simulink model "unit_decide"  (R2026b)
settings: Solver=FixedStepDiscrete  EnableMultiTasking=on
values from neighbouring files (symbols this model uses):
  STALL_SEC = 1.0    [sign_detector.sldd]
  VOTE_K = 3.0    [sign_detector.sldd]
  VOTE_N = 5.0    [sign_detector.sldd]
settings Model: DataDictionary=sign_detector.sldd  Creator=don  LastModifiedBy=don
settings SolverCC: PositivePriorityOrder=on
settings OptimizationCC: DifferentSizesBufferReuse=on  EfficientFloat2IntCast=on  EfficientTunableParamExpr=on  EnhancedBackFolding=on  LifeSpan=Inf  MaxStackSize=200000  OptimizationCustomize=off  OptimizeBlockOrder=speed  PassReuseOutputArgsAs=Individual arguments  UseDivisionForNetSlopeComputation=on
settings DebuggingCC: AlgebraicLoopMsg=error  ArtificialAlgebraicLoopMsg=error  AssertControl=DisableAll  BlockPriorityViolationMsg=error  BusObjectLabelMismatch=error  CheckMatrixSingularityMsg=error  InheritedTsInSrcMsg=error  IntegerOverflowMsg=error  IntegerSaturationMsg=error  ModelReferenceDataLoggingMessage=error  ModelReferenceIOMismatchMessage=error  NonBusSignalsTreatedAsBus=error  ParameterPrecisionLossMsg=error  ParameterTunabilityLossMsg=error  ParameterUnderflowMsg=error  ReadBeforeWriteMsg=EnableAllAsError  RootOutportRequireBusObject=error  SFcnCompatibilityMsg=error  SaveWithDisabledLinksMsg=error  SaveWithParameterizedLinksMsg=error  SigSpecEnsureSampleTimeMsg=error  SignalInfNanChecking=error  SignalLabelMismatchMsg=error  SignalRangeChecking=error  SolverPrmCheckMsg=error  StateNameClashWarn=warning  StrictBusMsg=ErrorOnBusTreatedAsVector  TasksWithSamePriorityMsg=error  UnconnectedInputMsg=error  UnconnectedLineMsg=error  UnconnectedOutputMsg=error  UnderSpecifiedDataTypeMsg=error  UniqueDataStoreMsg=error  UnknownTsInhSupMsg=error  UnnecessaryDatatypeConvMsg=warning  VariantConditionMismatch=error  VectorMatrixConversionMsg=error  WriteAfterReadMsg=EnableAllAsError  WriteAfterWriteMsg=EnableAllAsError
settings HardwareCC: ProdHWDeviceType=ARM Compatible->ARM Cortex-A (64-bit)  ProdLargestAtomicFloat=Double  ProdLargestAtomicInteger=LongLong  ProdLongLongMode=on
settings ModelReferenceCC: ModelReferenceNumInstancesAllowed=Single
settings SFSimCC: EnableRuntimeRecursion=off  MATLABDynamicMemAlloc=off
settings RTWCC: BuildConfiguration=Faster Runs  Description=Embedded Coder  HardwareBoard=Raspberry Pi (64bit)  SystemTargetFile=ert.tlc  TLCOptions="-aInlineSetEventsForThisBaseRateFcn=TLC_FALSE -aSuppressMultiTaskScheduler=TLC_FALSE  -aRateBasedStepFcn=0"  TargetLang=C++  TemplateMakefile=ert_default_tmf  Toolchain=GNU GCC RPIUtils
settings CodeAppCC: ForceParamTrailComments=on  IgnoreCustomStorageClasses=off  InsertBlockDesc=on  MATLABFcnDesc=on  MATLABSourceComments=on  OperatorAnnotations=on  ReqsInCode=on  SFDataObjDesc=on  SimulinkDataObjDesc=on  StateflowObjectComments=on
settings ERTTargetCC: CastingMode=Standards  CombineSignalStateStructs=on  EnableSignedLeftShifts=off  EnableSignedRightShifts=off  ExtModeIntrfLevel=Level2 - Open  ExtModeMexFile=ext_xcp  ExtModeStaticAlloc=on  GenerateSharedConstants=off  ParenthesesLevel=Standards  PreserveExpressionOrder=on  SubcomponentCodeInterfacePackaging=Nonreusable function  SupportNonFinite=off  SupportVariableSizeSignals=on  SuppressErrorStatus=on  TargetLangStandard=C++11 (ISO)  UtilityFuncGeneration=Shared location

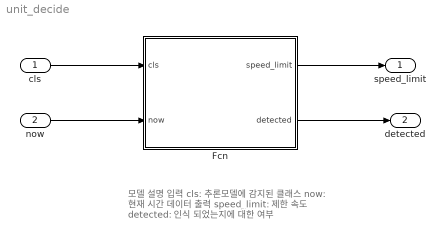
== system unit_decide ==
  note: 모델 설명
      | 입력
      | cls: 추론모델에 감지된 클래스
      | now: 현재 시간 데이터
      | 출력
      | speed_limit: 제한 속도
      | detected: 인식 되었는지에 대한 여부
  cls : Inport  OutDataTypeStr=double  PortDimensions=1  Interpolate=off
  now : Inport  Port=2  OutDataTypeStr=double  PortDimensions=1  Interpolate=off
  Fcn : MATLAB Function  TreatAsAtomicUnit=on
  speed_limit : Outport
  detected : Outport  Port=2
  wires:
  cls/1 -> Fcn/1(cls)
  now/1 -> Fcn/2(now)
  Fcn/1(speed_limit) -> speed_limit/1
  Fcn/2(detected) -> detected/1

== matlab function unit_decide/Fcn ==
  data: cls input double; speed_limit output double; now input double; detected output double; VOTE_N parameter double; VOTE_K parameter double; STALL_SEC parameter double
function [speed_limit, detected] = decide(cls, now, VOTE_N, VOTE_K, STALL_SEC)

TOL = 1e-9; % 시각 비교 오차 [초] (소수 합이 1.0보다 아주 조금 작게 나오는 것 보정)

persistent qc len prev_t limit
if isempty(qc)
    qc = zeros(VOTE_N, 1); % 최근 VOTE_N개 프레임의 클래스값
    len = 0;               % 큐에 든 값의 수
    prev_t = 0;            % 직전 프레임 시각
    limit = 0;             % 현재 제한속도 클래스
end

% 입력 정리: 클래스값이 0~4 정수가 아니면 0(표지판 없음)으로 봄 (cnt 배열 인덱스 보호)
if ~(cls >= 0 && cls <= 4 && cls == floor(cls))
    cls = 0;
end

% 인식 정지에서 벗어난 첫 프레임: 기록을 비우고 이 프레임부터 다시 셈 (SWR-02, SWR-32)
if len > 0 && now - prev_t >= STALL_SEC - TOL
    len = 0;
end
prev_t = now;

% 큐에 추가 (가득 찼으면 가장 오래된 값을 버림)
if len == VOTE_N
    qc(1:VOTE_N - 1) = qc(2:VOTE_N);
else
    len = len + 1;
end
qc(len) = cls;

% 확정 판단
detected = 0;
if len == VOTE_N
    cnt = zeros(4, 1);
    for i = 1:VOTE_N
        c = qc(i);
        if c > 0
            cnt(c) = cnt(c) + 1;
        end
    end
    for c = 1:4
        if cnt(c) >= VOTE_K
            detected = 1;
            limit = c; % 확정되면 제한속도 갱신, 확정이 풀려도 이전 값 유지 (SWR-03)
        end
    end
end

speed_limit = limit;
end
